simulink subsystem "Subsys_GFolConv_OuterCtrl_VDE4110"  (R2023b)
settings: Solver=VariableStepAuto  StartTime=0.0  StopTime=10.0  RelTol=1e-3
model mask{S_n=2e6, P_binst=1.5e6, f_n=50, T_LPF_P=33e-3, VDE4110_Pf_DBlow=49.8, VDE4110_Pf_DBhigh=50.2, VDE4110_Pf_droop=5, VDE4110_Pf_dPdt_max=1, VDE4110_Pf_isStorage=0, Q_ctrl_mode=3, T_PT1_Q=3.33, uq0ref=1, qmax=0.33, umax=1.04, deadband=0, p_pu=[0.1, 0.5, 0.6, 0.9, 1.0], q_pu=[0.0, 0.0, -0.05, -0.33, -0.33], p1=[0.94, 0.33], p2=[0.96, 0], p3=[1.04, 0], p4=[1.06, -0.33], cosphi_ref=1, Q_direction=0, T_s_ctrl=1e-3, datatype='double'}
  mask prompts: S_n "Nominal apparent power [VA]"; P_binst "Installed active power [W]"; f_n "Nominal frequency [Hz]"; T_LPF_P "Time constant of P(f) active power PT1 delay [s]"; VDE4110_Pf_DBlow "P(f) deadband lower limit [Hz]"; VDE4110_Pf_DBhigh "P(f) deadband higher limit [Hz]"; VDE4110_Pf_droop "P(f) droop [(df/f_n)/(dP/Pref)] [%]"; VDE4110_Pf_dPdt_max "P(f) maximum dP/dt [pu / s]"; VDE4110_Pf_isStorage "Generation unit is energy storage (1 = true, 0 = false)"; Q_ctrl_mode "Q-control mode (1 = Q(V), 2 = Q(P), 3 = Q(V) with deadband, 4 = cosphi)"; T_PT1_Q "Time constant of reactive power PT1 delay [s]"; uq0ref "U_Q0ref [pu]"; qmax "|Q_max| [pu]"; umax "U_max [pu]"; deadband "Voltage deadband [+- %]"; p_pu "P_grid points [pu]"; q_pu "Q_grid points [pu]"; p1 "P1 [V_grid, Q_grid] [pu]"; p2 "P2 [V_grid, Q_grid] [pu]"; p3 "P3 [V_grid, Q_grid] [pu]"; p4 "P4 [V_grid, Q_grid] [pu]"; cosphi_ref "cos(phi)"; Q_direction "Reactive power flow direction (1 = ind. Q injection, 0 = ind. Q consumption)"; T_s_ctrl "Controller sample time [s]"; datatype "Signal data type"
undefined symbols (not defined in the file): den_LPF_P, den_LPF_Q, num_LPF_P, num_LPF_Q
libraries: simulink x6
settings Model: Creator=winkens  LastModifiedBy=a.och
settings SolverCC: AlgebraicLoopSolver=TrustRegion
settings OptimizationCC: ReuseModelBlockBuffer=off
settings DebuggingCC: UnconnectedInputMsg=warning  UnconnectedOutputMsg=warning  UnconnectedLineMsg=warning
settings ModelReferenceCC: EnableRefExpFcnMdlSchedulingChecks=on
settings RTWCC: DLArmComputeVersion=19.05

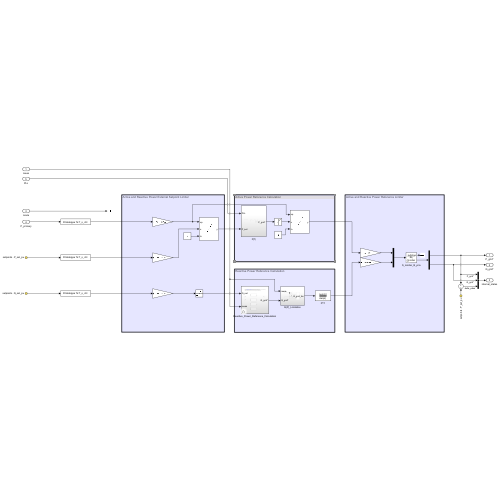
[thumbnail: Simulink's stored preview of the top-level diagram]
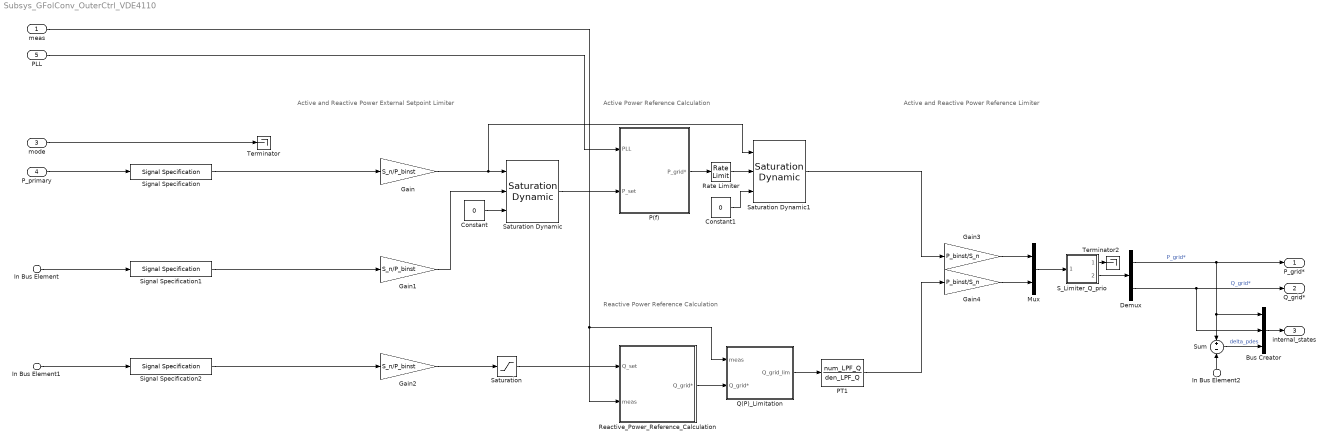
== system Subsys_GFolConv_OuterCtrl_VDE4110 ==
  note: Active and Reactive Power External Setpoint Limiter
  note: Active Power Reference Calculation
  note: Reactive Power Reference Calculation
  note: Active and Reactive Power Reference Limiter
  meas : Inport
  In Bus Element : Inport  Port=2  PortName=setpoints  Element=P_set_pu
  In Bus Element2 : Inport  Port=2  PortName=setpoints  Element=P_set_pu
  In Bus Element1 : Inport  Port=2  PortName=setpoints  Element=Q_set_pu
  mode : Inport  Port=3
  P_primary : Inport  Port=4
  PLL : Inport  Port=5
  Bus Creator : BusCreator  Inputs=3
  Constant : Constant  Value=0  OutDataTypeStr=datatype
  Constant1 : Constant  Value=0  OutDataTypeStr=datatype
  Demux : Demux  Outputs=2
  Gain : Gain  Gain=S_n/P_binst
  Gain1 : Gain  Gain=S_n/P_binst
  Gain2 : Gain  Gain=S_n/P_binst
  Gain3 : Gain  Gain=P_binst/S_n
  Gain4 : Gain  Gain=P_binst/S_n
  Mux : Mux  Inputs=2
  P(f) : Subsystem
  PT1 : DiscreteFilter  Numerator=num_LPF_Q  Denominator=den_LPF_Q  SampleTime=T_s_ctrl
  Q(P)_Limitation : Subsystem
  Rate Limiter : RateLimiter  RisingSlewLimit=VDE4110_Pf_dPdt_max  FallingSlewLimit=-VDE4110_Pf_dPdt_max  SampleTimeMode=inherited
  Reactive_Power_Reference_Calculation : Subsystem  Variant=on
  S_Limiter_Q_prio : Subsystem  ReferencedSubsystem=dq_Limiter  X_dq_max=1  datatype=datatype
  Saturation : Saturate  UpperLimit=0.33  LowerLimit=-0.33
  Saturation Dynamic : simulink/Discontinuities/Saturation Dynamic  OutMin=[]  OutMax=[]  OutDataTypeStr=Inherit: Same as second input  OutDataType=fixdt(1, 16)  OutScaling=2^-10  DoSatur=off
  Saturation Dynamic1 : simulink/Discontinuities/Saturation Dynamic  OutMin=[]  OutMax=[]  OutDataTypeStr=Inherit: Same as second input  OutDataType=fixdt(1, 16)  OutScaling=2^-10  DoSatur=off
  Signal Specification : SignalSpecification  OutDataTypeStr=datatype  SampleTime=T_s_ctrl
  Signal Specification1 : SignalSpecification  OutDataTypeStr=datatype  SampleTime=T_s_ctrl
  Signal Specification2 : SignalSpecification  OutDataTypeStr=datatype  SampleTime=T_s_ctrl
  Sum : Sum  Inputs=+|-
  Terminator : Terminator
  Terminator2 : Terminator
  P_grid* : Outport
  Q_grid* : Outport  Port=2
  internal_states : Outport  Port=3
  wires:
  Gain4/1 -> Mux/2
  Gain3/1 -> Mux/1
  Gain2/1 -> Saturation/1
  Gain1/1 -> Saturation Dynamic/2
  Gain/1 -> Saturation Dynamic1/1, Saturation Dynamic/1
  Q(P)_Limitation/1(Q_grid_lim) -> PT1/1
  Bus Creator/1 -> internal_states/1
  Demux/2 -> Q_grid*/1, Bus Creator/2  "Q_grid*"
  Demux/1 -> P_grid*/1, Bus Creator/1, Sum/1  "P_grid*"
  PT1/1 -> Gain4/1
  Saturation Dynamic1/1 -> Gain3/1
  Mux/1 -> S_Limiter_Q_prio/1
  S_Limiter_Q_prio/2 -> Demux/1
  S_Limiter_Q_prio/1 -> Terminator2/1
  mode/1 -> Terminator/1
  Constant1/1 -> Saturation Dynamic1/3
  Rate Limiter/1 -> Saturation Dynamic1/2
  P(f)/1(P_grid*) -> Rate Limiter/1
  Reactive_Power_Reference_Calculation/1(Q_grid*) -> Q(P)_Limitation/2(Q_grid*)
  meas/1 -> Reactive_Power_Reference_Calculation/2(meas), Q(P)_Limitation/1(meas)
  Saturation/1 -> Reactive_Power_Reference_Calculation/1(Q_set)
  P_primary/1 -> Signal Specification/1
  Saturation Dynamic/1 -> P(f)/2(P_set)
  Constant/1 -> Saturation Dynamic/3
  In Bus Element1/1 -> Signal Specification2/1
  In Bus Element/1 -> Signal Specification1/1
  PLL/1 -> P(f)/1(PLL)
  Signal Specification/1 -> Gain/1
  Signal Specification1/1 -> Gain1/1
  Signal Specification2/1 -> Gain2/1
  In Bus Element2/1 -> Sum/2
  Sum/1 -> Bus Creator/3  "delta_pdes"

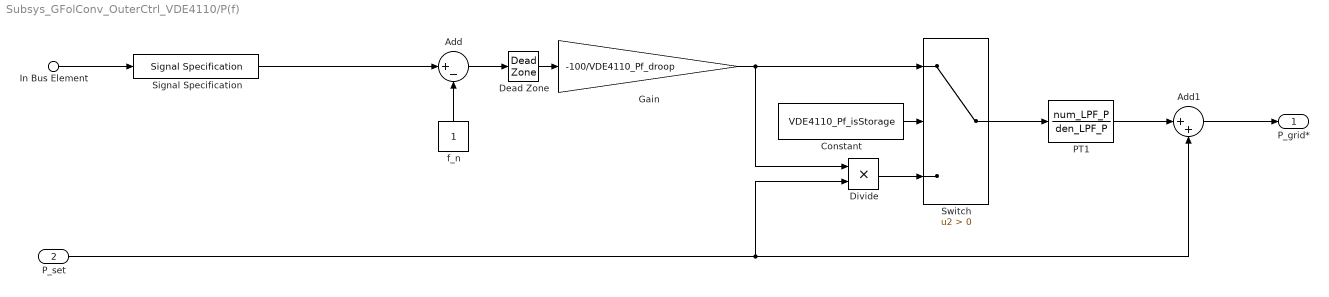
== system Subsys_GFolConv_OuterCtrl_VDE4110/P(f) ==
  In Bus Element : Inport  PortName=PLL  Element=f_PLL
  P_set : Inport  Port=2
  Add : Sum  Inputs=|+-
  Add1 : Sum  Inputs=|++
  Constant : Constant  Value=VDE4110_Pf_isStorage  OutDataTypeStr=datatype
  Dead Zone : DeadZone  LowerValue=(VDE4110_Pf_DBlow - f_n) / f_n  UpperValue=(VDE4110_Pf_DBhigh - f_n) / f_n
  Divide : Product  Inputs=**
  Gain : Gain  Gain=-100/VDE4110_Pf_droop
  PT1 : DiscreteFilter  Numerator=num_LPF_P  Denominator=den_LPF_P  SampleTime=T_s_ctrl
  Signal Specification : SignalSpecification  OutDataTypeStr=datatype  SampleTime=T_s_ctrl
  Switch : Switch  Criteria=u2 > Threshold  SaturateOnIntegerOverflow=off  InputSameDT=off
  f_n : Constant  OutDataTypeStr=datatype
  P_grid* : Outport
  wires:
  In Bus Element/1 -> Signal Specification/1
  Signal Specification/1 -> Add/1
  f_n/1 -> Add/2
  Add/1 -> Dead Zone/1
  Dead Zone/1 -> Gain/1
  P_set/1 -> Divide/2, Add1/2
  Add1/1 -> P_grid*/1
  Gain/1 -> Switch/1, Divide/1
  Constant/1 -> Switch/2
  Divide/1 -> Switch/3
  Switch/1 -> PT1/1
  PT1/1 -> Add1/1

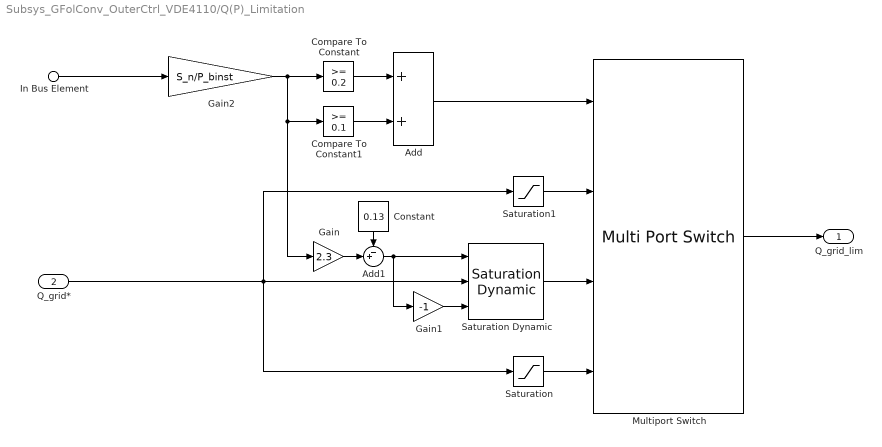
== system Subsys_GFolConv_OuterCtrl_VDE4110/Q(P)_Limitation ==
  In Bus Element : Inport  PortName=meas  Element=p_grid
  Q_grid* : Inport  Port=2
  Add : Sum
  Add1 : Sum  Inputs=-+|
  Compare To Constant : simulink/Logic and Bit Operations/Compare To Constant  relop=>=  const=0.2  OutDataTypeStr=uint8
  Compare To Constant1 : simulink/Logic and Bit Operations/Compare To Constant  relop=>=  const=0.1  OutDataTypeStr=uint8
  Constant : Constant  Value=0.13  OutDataTypeStr=datatype
  Gain : Gain  Gain=2.3
  Gain1 : Gain  Gain=-1
  Gain2 : Gain  Gain=S_n/P_binst
  Multiport Switch : MultiPortSwitch  DataPortOrder=Zero-based contiguous  zeroidx=on  SaturateOnIntegerOverflow=off  InputSameDT=off
  Saturation : Saturate  UpperLimit=0.33  LowerLimit=-0.33
  Saturation Dynamic : simulink/Discontinuities/Saturation Dynamic  OutMin=[]  OutMax=[]  OutDataTypeStr=Inherit: Same as second input  OutDataType=fixdt(1, 16)  OutScaling=2^-10  DoSatur=off
  Saturation1 : Saturate  UpperLimit=0.02  LowerLimit=-0.05
  Q_grid_lim : Outport
  wires:
  In Bus Element/1 -> Gain2/1
  Compare To Constant/1 -> Add/1
  Compare To Constant1/1 -> Add/2
  Add/1 -> Multiport Switch/1
  Saturation/1 -> Multiport Switch/4
  Saturation1/1 -> Multiport Switch/2
  Q_grid*/1 -> Saturation Dynamic/2, Saturation/1, Saturation1/1
  Multiport Switch/1 -> Q_grid_lim/1
  Saturation Dynamic/1 -> Multiport Switch/3
  Gain/1 -> Add1/2
  Constant/1 -> Add1/1
  Add1/1 -> Saturation Dynamic/1, Gain1/1
  Gain1/1 -> Saturation Dynamic/3
  Gain2/1 -> Gain/1, Compare To Constant1/1, Compare To Constant/1

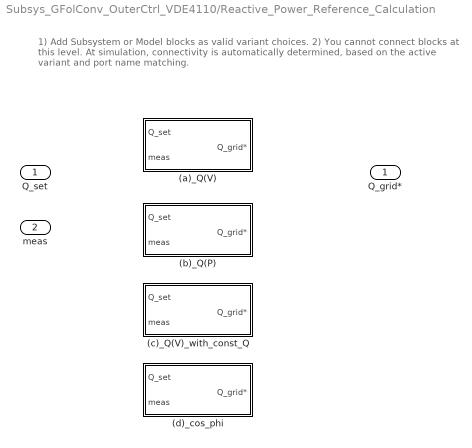
== system Subsys_GFolConv_OuterCtrl_VDE4110/Reactive_Power_Reference_Calculation ==
  note: 1) Add Subsystem or Model blocks as valid variant choices.
      | 2) You cannot connect blocks at this level. At simulation, connectivity is automatically
      | determined, based on the active variant and port name matching.
  Q_set : Inport
  meas : Inport  Port=2
  (a)_Q(V) : Subsystem  VariantControl=(default)
  (b)_Q(P) : Subsystem  VariantControl=Q_ctrl_mode == 2
  (c)_Q(V)_with_const_Q : Subsystem  VariantControl=Q_ctrl_mode == 3
  (d)_cos_phi : Subsystem  VariantControl=Q_ctrl_mode == 4
  Q_grid* : Outport

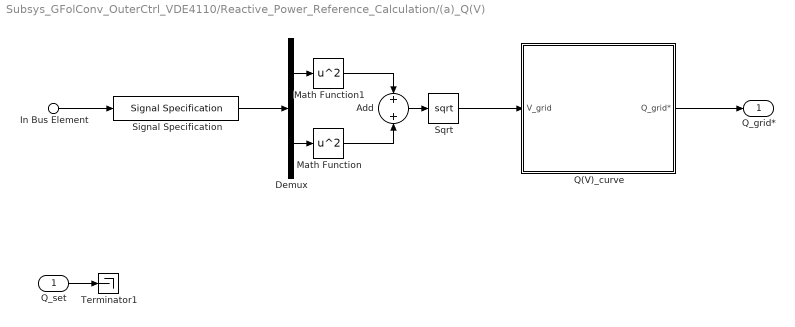
== system Subsys_GFolConv_OuterCtrl_VDE4110/Reactive_Power_Reference_Calculation/(a)_Q(V) ==
  Q_set : Inport
  In Bus Element : Inport  Port=2  PortName=meas  Element=dq+.v_grid_dq+
  Add : Sum  Inputs=+|+
  Demux : Demux  Outputs=2
  Math Function : Math  Operator=square
  Math Function1 : Math  Operator=square
  Q(V)_curve : Subsystem  mask{deadband=deadband, umax=umax, qmax=qmax, uq0ref=uq0ref}
      mask prompts: deadband "Voltage Deadband [+- %]"; umax "U_max [pu]"; qmax "|Q_max| [pu]"; uq0ref "U_Q0ref [pu]"
      mask DialogControl DescGroupVar Prompt: Q(V)-curve
      mask DialogControl DescTextVar Prompt: Q(V)-curve according to VDE 4110. Detailed parameter descriptions are given in the VDE 4110 document.
  Signal Specification : SignalSpecification  OutDataTypeStr=datatype  SampleTime=T_s_ctrl
  Sqrt : Sqrt
  Terminator1 : Terminator
  Q_grid* : Outport
  wires:
  In Bus Element/1 -> Signal Specification/1
  Q(V)_curve/1(Q_grid*) -> Q_grid*/1
  Demux/2 -> Math Function/1
  Demux/1 -> Math Function1/1
  Math Function1/1 -> Add/1
  Math Function/1 -> Add/2
  Add/1 -> Sqrt/1
  Sqrt/1 -> Q(V)_curve/1(V_grid)
  Q_set/1 -> Terminator1/1
  Signal Specification/1 -> Demux/1

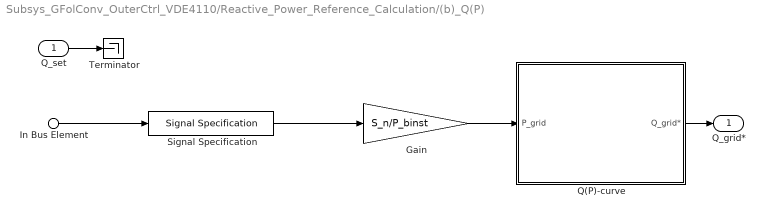
== system Subsys_GFolConv_OuterCtrl_VDE4110/Reactive_Power_Reference_Calculation/(b)_Q(P) ==
  Q_set : Inport
  In Bus Element : Inport  Port=2  PortName=meas  Element=p_grid
  Gain : Gain  Gain=S_n/P_binst
  Q(P)-curve : Subsystem  mask{q_pu=q_pu, p_pu=p_pu}
      mask prompts: q_pu "Q_grid points [pu]"; p_pu "P_grid points [pu]"
      mask DialogControl DescGroupVar Prompt: Q(P)-curve
      mask DialogControl DescTextVar Prompt: Q(P)-curve according to VDE 4110. Detailed parameter descriptions are given in the VDE 4110 document.
      mask DialogControl Control2 Prompt: In contrast to VDE 4110, here the active and reactive power values are given in active sign convention.
  Signal Specification : SignalSpecification  OutDataTypeStr=datatype  SampleTime=T_s_ctrl
  Terminator : Terminator
  Q_grid* : Outport
  wires:
  In Bus Element/1 -> Signal Specification/1
  Q_set/1 -> Terminator/1
  Q(P)-curve/1(Q_grid*) -> Q_grid*/1
  Gain/1 -> Q(P)-curve/1(P_grid)
  Signal Specification/1 -> Gain/1

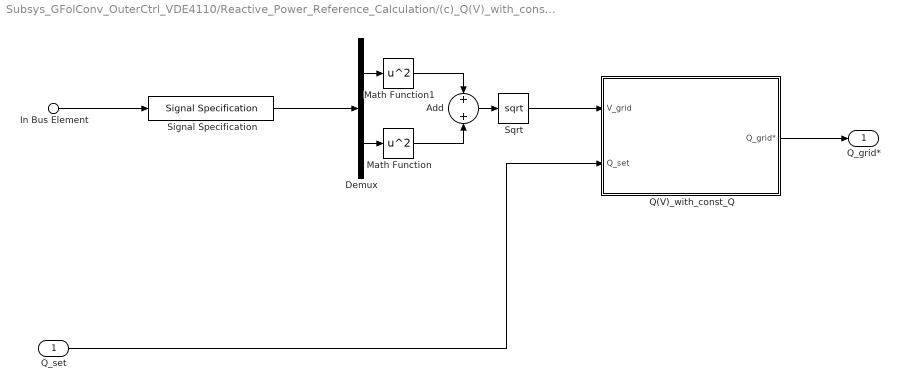
== system Subsys_GFolConv_OuterCtrl_VDE4110/Reactive_Power_Reference_Calculation/(c)_Q(V)_with_const_Q ==
  Q_set : Inport
  In Bus Element : Inport  Port=2  PortName=meas  Element=dq+.v_grid_dq+
  Add : Sum  Inputs=+|+
  Demux : Demux  Outputs=2
  Math Function : Math  Operator=square
  Math Function1 : Math  Operator=square
  Q(V)_with_const_Q : Subsystem  mask{p1=p1, p2=p2, p3=p3, p4=p4}
      mask prompts: p1 "P1 [V_grid, Q_grid] [pu]"; p2 "P2 [V_grid, Q_grid] [pu]"; p3 "P3 [V_grid, Q_grid] [pu]"; p4 "P4 [V_grid, Q_grid] [pu]"
      mask DialogControl DescGroupVar Prompt: Constant Q with voltage limitation
      mask DialogControl DescTextVar Prompt: Q(V)-curve according to VDE 4110. Detailed parameter descriptions are given in the VDE 4110 document.
      mask DialogControl Control2 Prompt: In contrast to VDE 4110, here the reactive power values are given in active sign convention.
  Signal Specification : SignalSpecification  OutDataTypeStr=datatype  SampleTime=T_s_ctrl
  Sqrt : Sqrt
  Q_grid* : Outport
  wires:
  In Bus Element/1 -> Signal Specification/1
  Q_set/1 -> Q(V)_with_const_Q/2(Q_set)
  Demux/1 -> Math Function1/1
  Add/1 -> Sqrt/1
  Math Function1/1 -> Add/1
  Math Function/1 -> Add/2
  Demux/2 -> Math Function/1
  Sqrt/1 -> Q(V)_with_const_Q/1(V_grid)
  Q(V)_with_const_Q/1(Q_grid*) -> Q_grid*/1
  Signal Specification/1 -> Demux/1

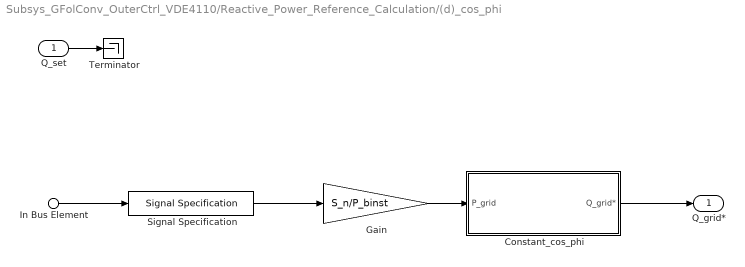
== system Subsys_GFolConv_OuterCtrl_VDE4110/Reactive_Power_Reference_Calculation/(d)_cos_phi ==
  Q_set : Inport
  In Bus Element : Inport  Port=2  PortName=meas  Element=p_grid
  Constant_cos_phi : Subsystem  mask{cosphi_ref=cosphi_ref, inductive_Q_infeed=Q_direction}
      mask prompts: cosphi_ref "cos(phi)"; inductive_Q_infeed "Reactive power flow direction (1 = ind. Q injection, 0 = ind. Q consumption)"
      mask DialogControl DescGroupVar Prompt: Constant cos(phi)
      mask DialogControl DescTextVar Prompt: Constant cos(phi) behavior according to VDE 4110. Detailed parameter descriptions are given in the VDE 4110 document.
  Gain : Gain  Gain=S_n/P_binst
  Signal Specification : SignalSpecification  OutDataTypeStr=datatype  SampleTime=T_s_ctrl
  Terminator : Terminator
  Q_grid* : Outport
  wires:
  In Bus Element/1 -> Signal Specification/1
  Q_set/1 -> Terminator/1
  Constant_cos_phi/1(Q_grid*) -> Q_grid*/1
  Gain/1 -> Constant_cos_phi/1(P_grid)
  Signal Specification/1 -> Gain/1

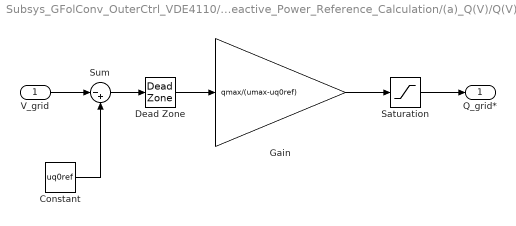
== system Subsys_GFolConv_OuterCtrl_VDE4110/Reactive_Power_Reference_Calculation/(a)_Q(V)/Q(V)_curve ==
  V_grid : Inport
  Constant : Constant  Value=uq0ref  OutDataTypeStr=datatype
  Dead Zone : DeadZone  LowerValue=-deadband/100  UpperValue=+deadband/100
  Gain : Gain  Gain=qmax/(umax-uq0ref)
  Saturation : Saturate  UpperLimit=qmax  LowerLimit=-qmax
  Sum : Sum  Inputs=|-+
  Q_grid* : Outport  VectorParamsAs1DForOutWhenUnconnected=off
  wires:
  V_grid/1 -> Sum/1
  Sum/1 -> Dead Zone/1
  Gain/1 -> Saturation/1
  Dead Zone/1 -> Gain/1
  Saturation/1 -> Q_grid*/1
  Constant/1 -> Sum/2

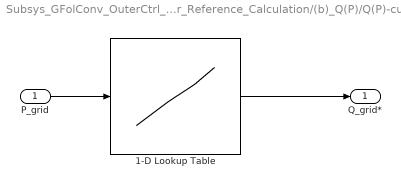
== system Subsys_GFolConv_OuterCtrl_VDE4110/Reactive_Power_Reference_Calculation/(b)_Q(P)/Q(P)-curve ==
  P_grid : Inport
  1-D Lookup Table : Lookup_n-D  NumberOfTableDimensions=1  BreakpointsForDimension1=p_pu  Table=q_pu  InternalRulePriority=Speed  RndMeth=Simplest
  Q_grid* : Outport  VectorParamsAs1DForOutWhenUnconnected=off
  wires:
  P_grid/1 -> 1-D Lookup Table/1
  1-D Lookup Table/1 -> Q_grid*/1

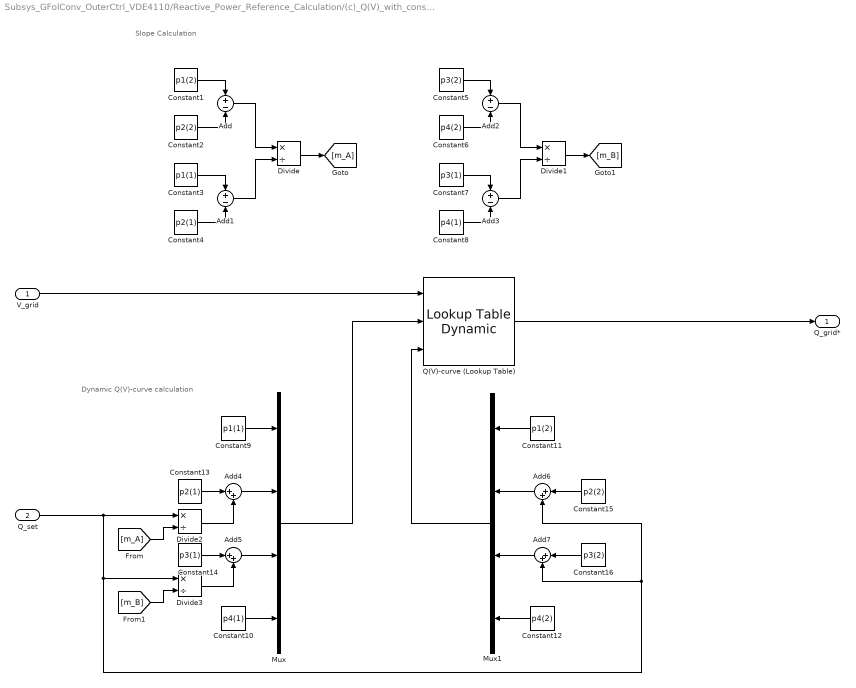
== system Subsys_GFolConv_OuterCtrl_VDE4110/Reactive_Power_Reference_Calculation/(c)_Q(V)_with_const_Q/Q(V)_with_const_Q ==
  note: Dynamic Q(V)-curve calculation
  note: Slope Calculation
  V_grid : Inport
  Q_set : Inport  Port=2
  Add{,1..3} (4 alike) : Sum  Inputs=+|-
  Add{4..7} (4 alike) : Sum  Inputs=|++
  Constant1 : Constant  Value=p1(2)  OutDataTypeStr=datatype
  Constant10 : Constant  Value=p4(1)  OutDataTypeStr=datatype
  Constant11 : Constant  Value=p1(2)  OutDataTypeStr=datatype
  Constant12 : Constant  Value=p4(2)  OutDataTypeStr=datatype
  Constant13 : Constant  Value=p2(1)  OutDataTypeStr=datatype
  Constant14 : Constant  Value=p3(1)  OutDataTypeStr=datatype
  Constant15 : Constant  Value=p2(2)  OutDataTypeStr=datatype
  Constant16 : Constant  Value=p3(2)  OutDataTypeStr=datatype
  Constant2 : Constant  Value=p2(2)  OutDataTypeStr=datatype
  Constant3 : Constant  Value=p1(1)  OutDataTypeStr=datatype
  Constant4 : Constant  Value=p2(1)  OutDataTypeStr=datatype
  Constant5 : Constant  Value=p3(2)  OutDataTypeStr=datatype
  Constant6 : Constant  Value=p4(2)  OutDataTypeStr=datatype
  Constant7 : Constant  Value=p3(1)  OutDataTypeStr=datatype
  Constant8 : Constant  Value=p4(1)  OutDataTypeStr=datatype
  Constant9 : Constant  Value=p1(1)  OutDataTypeStr=datatype
  Divide{,1..3} (4 alike) : Product  Inputs=*/
  Mux : Mux
  Mux1 : Mux
  Q(V)-curve (Lookup Table) : simulink/Lookup Tables/Lookup Table Dynamic  LookUpMeth=Interpolation-Use End Values  OutDataType=datatype  OutScaling=[]  OutputDataTypeScalingMode=Specify via dialog  OutDataTypeStr=datatype  DoSatur=off
  Q_grid* : Outport  VectorParamsAs1DForOutWhenUnconnected=off
  wires:
  V_grid/1 -> Q(V)-curve (Lookup Table)/1
  Q(V)-curve (Lookup Table)/1 -> Q_grid*/1
  Constant1/1 -> Add/1
  Constant2/1 -> Add/2
  Constant4/1 -> Add1/2
  Constant3/1 -> Add1/1
  Add/1 -> Divide/1
  Add1/1 -> Divide/2
  Divide/1 -> [m_A]
  Divide1/1 -> [m_B]
  Constant7/1 -> Add3/1
  Add2/1 -> Divide1/1
  Constant8/1 -> Add3/2
  Add3/1 -> Divide1/2
  Constant6/1 -> Add2/2
  Constant5/1 -> Add2/1
  Constant9/1 -> Mux/1
  Constant10/1 -> Mux/4
  Mux/1 -> Q(V)-curve (Lookup Table)/2
  Mux1/1 -> Q(V)-curve (Lookup Table)/3
  Constant11/1 -> Mux1/1
  Constant12/1 -> Mux1/4
  Add5/1 -> Mux/3
  Add4/1 -> Mux/2
  Constant13/1 -> Add4/1
  Constant14/1 -> Add5/1
  Divide2/1 -> Add4/2
  Divide3/1 -> Add5/2
  [m_A] -> Divide2/2
  [m_B] -> Divide3/2
  Add6/1 -> Mux1/2
  Add7/1 -> Mux1/3
  Constant16/1 -> Add7/1
  Constant15/1 -> Add6/1
  Q_set/1 -> Add7/2, Add6/2, Divide3/1, Divide2/1

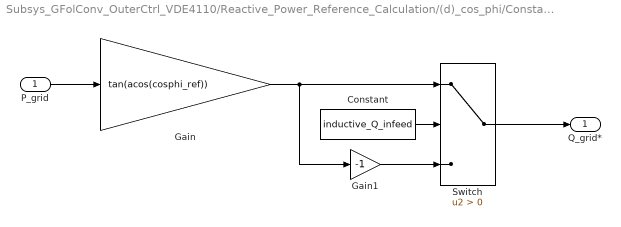
== system Subsys_GFolConv_OuterCtrl_VDE4110/Reactive_Power_Reference_Calculation/(d)_cos_phi/Constant_cos_phi ==
  P_grid : Inport
  Constant : Constant  Value=inductive_Q_infeed  OutDataTypeStr=datatype
  Gain : Gain  Gain=tan(acos(cosphi_ref))
  Gain1 : Gain  Gain=-1
  Switch : Switch  Criteria=u2 > Threshold  SaturateOnIntegerOverflow=off  InputSameDT=off
  Q_grid* : Outport  VectorParamsAs1DForOutWhenUnconnected=off
  wires:
  Gain/1 -> Gain1/1, Switch/1
  P_grid/1 -> Gain/1
  Constant/1 -> Switch/2
  Gain1/1 -> Switch/3
  Switch/1 -> Q_grid*/1
